simulink model "VFD_final"  (R2025b)
settings: Solver=VariableStepAuto  StartTime=0.0  StopTime=10  RelTol=1e-3
libraries: ee_lib x18, fl_lib x9, nesl_utility x8, eePwmGeneratorTwoLevel x1, dspstat3 x1, eeSinGeneratorThreePhase x1, simulink x1
settings Model: Creator=Administrator  LastModifiedBy=WELCOME
settings SolverCC: AlgebraicLoopSolver=TrustRegion
settings DebuggingCC: UnconnectedInputMsg=warning  UnconnectedOutputMsg=warning  UnconnectedLineMsg=warning
settings ModelReferenceCC: EnableRefExpFcnMdlSchedulingChecks=on
settings SFSimCC: CustomCodeUndefinedFunction=UseInterfaceOnly
settings RTWCC: GPUComputeCapability=3.5  DLArmComputeVersion=19.05

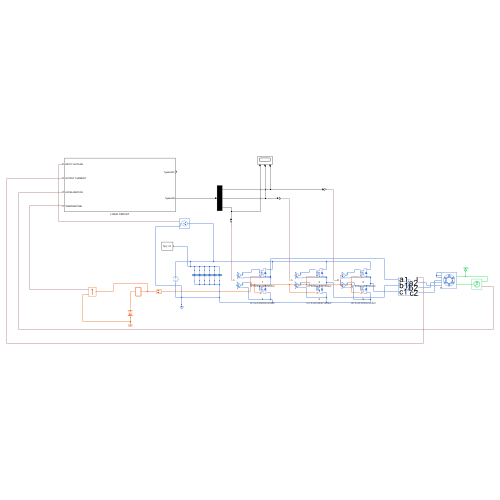
[thumbnail: Simulink's stored preview of the top-level diagram]
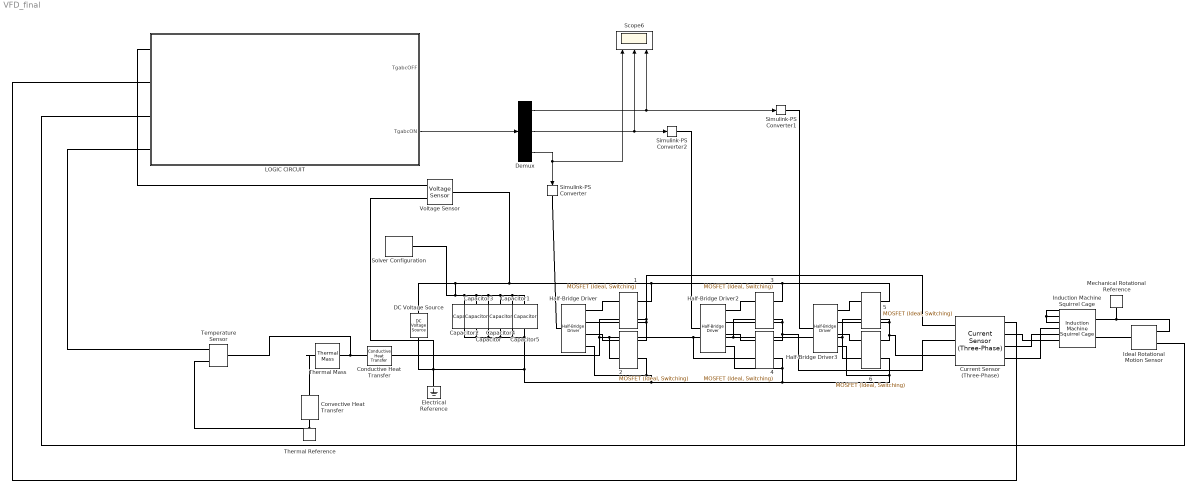
== system VFD_final ==
  {1..6} (6 alike) : ee_lib/Semiconductors & Converters/MOSFET (Ideal, Switching)  PartSpecification="{\"CollectionId\":\"SimscapeElectrical\",\"CollectionVersion\":\"1.0.0\",\"DatasetId\":\"IXYS|IXFN50N120SiC|simscape.electrical.mosfetIdealSwitching\",\"DisplayName\":\"IXYS:IXFN50N120SiC\"}"  port_option=ee.enum.controlport.elec  Rds=0.044 % Datasheet derived Ohm  Goff=2e-09 % Datasheet derived 1/Ohm  Vth=2.6 % Datasheet derived V  diode_param=ee.enum.semiconductors.protectionDiode.nodynamics  diode_Vf=2.21 % Datasheet derived V  diode_Ron=0.015 % Datasheet derived Ohm  diode_Goff=1e-05 % Library default 1/Ohm  diode_C=50e-9 % Parameter not set F  diode_iRM=-235 % Parameter not set A  diode_iF=300 % Parameter not set A  diode_idot=-50 % Parameter not set A/us  diode_trr_param=ee.enum.converters.diodeReverseParam.trr_factor  diode_trr_factor=3 % Parameter not set  diode_trr=15 % Parameter not set us  diode_Qrr=1500 % Parameter not set s*uA  ids_specify=off  ids_priority=None  ids=0 A  ids_nominal_specify=off  ids_nominal_value=1  ids_nominal_unit=A  vds_specify=off  vds_priority=None  vds=0 V  vds_nominal_specify=off  vds_nominal_value=1  vds_nominal_unit=V  vgs_specify=off  vgs_priority=None  vgs=0 V  vgs_nominal_specify=off  vgs_nominal_value=1  vgs_nominal_unit=V  thermal_loss_option=ee.enum.converters.thermalLossOption.tabulated2d  Von_data=[0 0.16 0.32 0.48 0.64 0.81 0.98 1.15 1.33 1.52 1.73 1.93 2.14 2.35 2.59 2.84 3.1 3.35 3.61 3.92 4.24 4.55 4.89 5.23;0 0.29 0.58 0.87 1.16 1.5 1.84 2.18 2.53 2.9 3.28 3.66 4.07 4.5 4.93 5.37 5.8 6.37 6.96 7.55 8.2 8.92 9.63 10.35] % Datasheet derived V  Tj=[25 150] % Datasheet derived degC  Iout_data=[0 4.33 8.67 13 17.34 21.67 26 30.34 34.67 39 43.34 47.67 52.01 56.34 60.67 65.01 69.34 73.68 78.01 82.34 86.68 91.01 95.35 99.68] % Datasheet derived A  Eon_data=[0.11 0.15 0.19 0.22 0.26 0.3 0.34 0.38 0.41 0.45 0.49 0.53 0.56 0.6 0.64 0.68 0.71 0.75 0.79 0.83 0.86 0.9 0.94 0.98 1.01 1.05 1.09 1.13 1.17 1.21 1.25 1.29 1.33 1.38 1.42 1.46 1.5 1.55 1.59 1.63 1.67 1.72 1.76 1.8 1.85 1.9 1.94 1.99 2.04 2.09 2.13 2.18 2.23 2.27 2.32 2.37 2.42 2.46 2.51 2.56 2.6 2.65 2.69 2.74 2.78 2.83 2.87 2.92 2.96 3.01 3.05 3.1] % Datasheet derived mJ  Eoff_data=[0 0.02 0.01 0 0.01 0.02 0.03 0.04 0.05 0.06 0.07 0.08 0.09 0.1 0.11 0.12 0.13 0.14 0.15 0.16 0.17 0.18 0.19 0.2 0.22 0.23 0.24 0.25 0.26 0.27 0.29 0.3 0.31 0.32 0.33 0.34 0.35 0.37 0.38 0.39 0.4 0.41 0.43 0.44 0.45 0.46 0.47 0.48 0.5 0.51 0.52 0.53 0.55 0.56 0.57 0.59 0.6 0.61 0.63 0.64 0.65 0.67 0.68 0.7 0.71 0.73 0.74 0.75 0.77 0.78 0.8 0.81] % Datasheet derived mJ  Eon_data_3D=[zeros(2, 5, 3)] % Parameter not set J  Eoff_data_3D=[zeros(2, 5, 3)] % Parameter not set J  Tj_loss=150 % Datasheet derived degC  Iout_data_loss=[0 1.12 2.23 3.35 4.47 5.58 6.7 7.81 8.93 10.05 11.16 12.28 13.4 14.51 15.63 16.75 17.86 18.98 20.09 21.21 22.33 23.44 24.56 25.68 26.79 27.91 29.02 30.14 31.26 32.37 33.49 34.61 35.72 36.84 37.96 39.07 40.19 41.3 42.42 43.54 44.65 45.77 46.89 48 49.12 50.24 51.35 52.47 53.58 54.7 55.82 56.93 58.05 59.17 60.28 61.4 62.51 63.63 64.75 65.86 66.98 68.1 69.21 70.33 71.45 72.56 73.68 74.79 75.91 77.03 78.14 79.26] % Datasheet derived A  tabulateWithVds=false % Parameter not set  Vds_loss=[0, 150, 300] % Parameter not set V  Eon_scalar=22.86e-3 % Parameter not set J  Eoff_scalar=17.14e-3 % Parameter not set J  Voff=800 % Datasheet derived V  Iout_scalar=600 % Parameter not set A  useCurrentFromPreviousCycle=false % Parameter not set  useVoltageFromPreviousCycle=false % Parameter not set  diodeModelType=ee.enum.converters.diodeModelType.tabulated  diodeTableType=ee.enum.diode.tableType.IfMat  diode_ReverseIVType=ee.enum.diode.diodeReverseIV.constant  diode_IfMat=[0 0.2663 0.5658 2.7227 13.8624 40.5914 79.6704 138.41;0 0.3166 0.63 4.3646 25.9282 65.8936 119.1956 183.5255] % Datasheet derived A  diode_VfMat=[.9, 1.15, 1.25, 1.5, 1.75, 2.17, 2.6, 2.85; .58, .68, .75, 1.1, 1.38, 1.77, 2.27, 2.7] % Parameter not set V  diode_TjVec=[25 150] % Datasheet derived degC  diode_VfVec=[0 1.05 2.1 3.15 4.19 5.24 6.29 7.34] % Datasheet derived V  diode_IfVec=[.1, .2, .5, 1, 2, 4, 7, 10] % Parameter not set A  diode_IrMat=[1e-06, 2e-06, 5e-06, 1e-05, 2.5e-05, 5e-05, .0001; 2e-06, 5e-06, 1e-05, 4e-05, 8e-05, .0002, .0005] % Parameter not set A  diode_VrMat=[10, 100, 200, 250, 300, 325, 350; 10, 70, 160, 220, 270, 300, 320] % Parameter not set V  diode_VrVec=[10, 20, 40, 50, 70, 80, 100] % Parameter not set V  diode_IrVec=[1e-06, 2e-06, 5e-06, 1e-05, 2e-05, 5e-05, .0001] % Parameter not set A  diode_Vr=-600 % Parameter not set V  diode_Ls=150 % Parameter not set nH  diode_Erec=0.03 % Parameter not set J  diode_rec_loss_model=ee.enum.diode.reverseRecoveryModel.fixed  diode_ErecVal=0 % Parameter not set J  diode_scaleWithIandV=true % Parameter not set  diode_ErecMat=zeros(2, 3) % Parameter not set J  diode_TjrecVec=[298.15, 398.15] % Parameter not set K  diode_IfrecVec=[.1, 1, 10] % Parameter not set A  diode_IrecVal=10 % Parameter not set A  diode_VrecVal=10 % Parameter not set V  diode_tFilter=1 / 1000 / 100 % Parameter not set s  separateThermalPortForDiode=false % Parameter not set  thermal_network_parameterization=ee.enum.thermalNetworkTopology.external  Rth=[.03, .2] % Parameter not set K/W  Rth_Cauer=[.03, .1, .2] % Parameter not set K/W  Rth_Foster=[.08, .14, .22, .16] % Parameter not set K/W  thermal_mass_parameterization=ee.enum.thermalNetwork.timeconstant  thermal_mass=[3, 25] % Parameter not set J/K  thermal_mass_Cauer=[3, 10, 25] % Parameter not set J/K  thermal_mass_Foster=[.001, .005, .05, .5] % Parameter not set J/K  thermal_time_constant=[.1, 5] % Parameter not set s  thermal_time_constant_Cauer=[.1, 1, 5] % Parameter not set s  thermal_time_constant_Foster=[7e-05, .0007, .01, .08] % Parameter not set s  thermal_mass_initial_temperatures=[25, 25] % Parameter not set degC  thermal_mass_initial_temperatures_Cauer=[25, 25, 25] % Parameter not set degC  junction_thermal_mass=19.4 % Datasheet derived J/K  Tvec_initial_Foster=[25, 25, 25, 25] % Parameter not set degC  RthDiode=[.03, .2] % Parameter not set K/W  RthCauerDiode=[.03, .1, .2] % Parameter not set K/W  RthFosterDiode=[.03, .2] % Parameter not set K/W  thermalMassDiode=[3, 25] % Parameter not set J/K  thermalMassCauerDiode=[3, 10, 25] % Parameter not set J/K  thermalMassFosterDiode=[33, 50] % Parameter not set J/K  thermalTauDiode=[.1, 5] % Parameter not set s  thermalTauCauerDiode=[.1, 1, 5] % Parameter not set s  thermalTauFosterDiode=[1, 10] % Parameter not set s  thermalMassInitTempDiode=[25, 25] % Parameter not set degC  thermalMassInitTempCauerDiode=[25, 25, 25] % Parameter not set degC  junctionthermalMassDiode=0.1 % Parameter not set J/K  TVecInitialFosterDiode=[25, 25, 25, 25] % Parameter not set degC  no_thermal_network=0 % Parameter not set  mosfet_junction_temperature_specify=off  mosfet_junction_temperature_priority=None  mosfet_junction_temperature=25 degC  mosfet_junction_temperature_nominal_specify=off  mosfet_junction_temperature_nominal_value=1  mosfet_junction_temperature_nominal_unit=degC  diode_junction_temperature_specify=off  diode_junction_temperature_priority=None  diode_junction_temperature=25 degC  diode_junction_temperature_nominal_specify=off  diode_junction_temperature_nominal_value=1  diode_junction_temperature_nominal_unit=degC  Qj_specify=off  Qj_priority=None  Qj=0 W  Qj_nominal_specify=off  Qj_nominal_value=1  Qj_nominal_unit=W  accumulatedSwitchingLosses_specify=off  accumulatedSwitchingLosses_priority=None  accumulatedSwitchingLosses=0 J
      settings: AttributesFormatString=IXYS:IXFN50N120SiC  InternalSimscapePortConfiguration="{\"Bottom\":[],\"Left\":[{\"id\":\"G_elec\",\"label\":\"\",\"type\":\"foundation.electrical.electrical\"},{\"id\":\"H\",\"label\":\"\",\"type\":\"foundation.thermal.thermal\"}],\"Right\":[{\"id\":\"D\",\"label\":\"\",\"type\":\"foundation.electrical.electrical\"},{\"id\":\"S\",\"label\":\"\",\"type\":\"foundation.electrical.electrical\"}],\"Top\":[]}"
  Capacitor{,1..5} (6 alike) : ee_lib/Passive/Capacitor  cap_option=ee.enum.passive.capacitor.capOption.const  c=550e-6 F  Cvec=[1e-05, 1e-06] F  Vvec=[0, 10] V  CV_table_symmetry=ee.enum.passive.capacitor.tableSymmetry.yes  f_vec=[1, 10] kHz  DFext_vec=[.8, 1.2]  enable_C_tol=ee.enum.toleranceApplication.none  averaging_period=0 s  C_tol=5  tol_distribution=ee.enum.toleranceDistribution.uniform  nSigma=4  r=1 Ohm  g=0 1/Ohm  enable_operating_limits=ee.enum.enable.no  operating_limit_action=ee.enum.passive.reportOpLim.warn  max_working_voltage_range=[-25, 25] V  power_rating=1 W  maxTemperature=85 degC  thermalEnable=false  thermalMass=1 J/K  i_specify=off  i_priority=None  i=0 A  i_nominal_specify=off  i_nominal_value=1  i_nominal_unit=A  v_specify=on  v_priority=None  v=565 V  v_nominal_specify=off  v_nominal_value=1  v_nominal_unit=V  vc_specify=off  vc_priority=High  vc=0 V  vc_nominal_specify=off  vc_nominal_value=1  vc_nominal_unit=V  T_specify=off  T_priority=None  T=298.15 K  T_nominal_specify=off  T_nominal_value=1  T_nominal_unit=K
  Conductive Heat Transfer : fl_lib/Thermal/Thermal Elements/Conductive Heat Transfer  thermal_type=foundation.enum.ConstantVariableTabulated.Constant  wall_geometry=foundation.enum.ConductionWallGeometry.Planar  area=20e-4 m^2  thickness=0.3 m  d_in=0.05 m  d_out=0.1 m  L=1 m  th_cond_min=10 W/(K*m)  th_cond=5 W/(K*m)  th_cond_TLU=[413, 401, 392, 383, 371, 357, 342] W/(K*m)  temp_TLU=[200, 273, 400, 600, 800, 1000, 1200] K  T_specify=off  T_priority=None  T=0 K  T_nominal_specify=off  T_nominal_value=1  T_nominal_unit=K  Q_specify=off  Q_priority=None  Q=0 W  Q_nominal_specify=off  Q_nominal_value=1  Q_nominal_unit=W
  Convective Heat Transfer : fl_lib/Thermal/Thermal Elements/Convective Heat Transfer  thermal_type=foundation.enum.constant_variable.constant  area=1e-4 m^2  heat_tr_coeff=20 W/(K*m^2)  min_heat_tr_coeff=1e-3 W/(K*m^2)  T_specify=off  T_priority=None  T=0 K  T_nominal_specify=off  T_nominal_value=1  T_nominal_unit=K  Q_specify=off  Q_priority=None  Q=0 W  Q_nominal_specify=off  Q_nominal_value=1  Q_nominal_unit=W
  Current Sensor (Three-Phase) : ee_lib/Sensors & Transducers/Current Sensor (Three-Phase)
      settings: InternalSimscapePortConfiguration="{\"Bottom\":[],\"Left\":[{\"id\":\"a1\",\"label\":\"a1\",\"type\":\"foundation.electrical.electrical\"},{\"id\":\"b1\",\"label\":\"b1\",\"type\":\"foundation.electrical.electrical\"},{\"id\":\"c1\",\"label\":\"c1\",\"type\":\"foundation.electrical.electrical\"}],\"Right\":[{\"id\":\"I_output\",\"label\":\"I\",\"type\":\"output\"},{\"id\":\"a2\",\"label\":\"a2\",\"type\":\"foundation.electrical.electrical\"},{\"id\":\"b2\",\"label\":\"b2\",\"type\":\"foundation.electrical.electrical\"},{\"id\":\"c2\",\"label\":\"c2\",\"type\":\"foundation.electrical.electrical\"}],\"Top\":[]}"
  DC Voltage Source : ee_lib/Additional Components/SPICE Sources/DC Voltage Source  DC=650 V
  Demux : Demux  Outputs=3
  Electrical Reference : fl_lib/Electrical/Electrical Elements/Electrical Reference
  Half-Bridge Driver : ee_lib/Semiconductors & Converters/Half-Bridge Driver  port_option=ee.enum.controlport.ps  uHigh=2.0 V  uLow=0.8 V  uHighValue=3  uLowValue=0.3  vHigh=22 V  vLow=-3 V  tpLH=50 ns  tdLH=100 ns  tpHL=50 ns  tdHL=100 ns  parameterization=ee.enum.semiconductors.gateDriverParam.outputImpedance  rHigh=2 Ohm  rLow=2 Ohm  tRise=20 ns  tFall=20 ns  cLoad=10 nF  ZonTime_specify=off  ZonTime_priority=None  ZonTime=0 s  ZoffTime_specify=off  ZoffTime_priority=None  ZoffTime=0 s  power_dissipated_high_side_specify=off  power_dissipated_high_side_priority=None  power_dissipated_high_side=0 W  power_dissipated_high_side_nominal_specify=off  power_dissipated_high_side_nominal_value=1  power_dissipated_high_side_nominal_unit=W  power_dissipated_low_side_specify=off  power_dissipated_low_side_priority=None  power_dissipated_low_side=0 W  power_dissipated_low_side_nominal_specify=off  power_dissipated_low_side_nominal_value=1  power_dissipated_low_side_nominal_unit=W
      settings: InternalSimscapePortConfiguration="{\"Bottom\":[],\"Left\":[{\"id\":\"u\",\"label\":\"u\",\"type\":\"input\"}],\"Right\":[{\"id\":\"HO\",\"label\":\"HO\",\"type\":\"foundation.electrical.electrical\"},{\"id\":\"HS\",\"label\":\"HS\",\"type\":\"foundation.electrical.electrical\"},{\"id\":\"LO\",\"label\":\"LO\",\"type\":\"foundation.electrical.electrical\"},{\"id\":\"LS\",\"label\":\"LS\",\"type\":\"foundation.electrical.electrical\"}],\"Top\":[]}"
  Half-Bridge Driver2 : ee_lib/Semiconductors & Converters/Half-Bridge Driver  port_option=ee.enum.controlport.ps  uHigh=2.0 V  uLow=0.8 V  uHighValue=3  uLowValue=0.3  vHigh=22 V  vLow=-3 V  tpLH=50 ns  tdLH=100 ns  tpHL=50 ns  tdHL=100 ns  parameterization=ee.enum.semiconductors.gateDriverParam.outputImpedance  rHigh=2 Ohm  rLow=2 Ohm  tRise=20 ns  tFall=20 ns  cLoad=10 nF  ZonTime_specify=off  ZonTime_priority=None  ZonTime=0 s  ZoffTime_specify=off  ZoffTime_priority=None  ZoffTime=0 s  power_dissipated_high_side_specify=off  power_dissipated_high_side_priority=None  power_dissipated_high_side=0 W  power_dissipated_high_side_nominal_specify=off  power_dissipated_high_side_nominal_value=1  power_dissipated_high_side_nominal_unit=W  power_dissipated_low_side_specify=off  power_dissipated_low_side_priority=None  power_dissipated_low_side=0 W  power_dissipated_low_side_nominal_specify=off  power_dissipated_low_side_nominal_value=1  power_dissipated_low_side_nominal_unit=W
      settings: InternalSimscapePortConfiguration="{\"Bottom\":[],\"Left\":[{\"id\":\"u\",\"label\":\"u\",\"type\":\"input\"}],\"Right\":[{\"id\":\"HO\",\"label\":\"HO\",\"type\":\"foundation.electrical.electrical\"},{\"id\":\"HS\",\"label\":\"HS\",\"type\":\"foundation.electrical.electrical\"},{\"id\":\"LO\",\"label\":\"LO\",\"type\":\"foundation.electrical.electrical\"},{\"id\":\"LS\",\"label\":\"LS\",\"type\":\"foundation.electrical.electrical\"}],\"Top\":[]}"
  Half-Bridge Driver3 : ee_lib/Semiconductors & Converters/Half-Bridge Driver  port_option=ee.enum.controlport.ps  uHigh=2.0 V  uLow=0.8 V  uHighValue=3  uLowValue=0.3  vHigh=22 V  vLow=-3 V  tpLH=50 ns  tdLH=100 ns  tpHL=50 ns  tdHL=100 ns  parameterization=ee.enum.semiconductors.gateDriverParam.outputImpedance  rHigh=2 Ohm  rLow=2 Ohm  tRise=20 ns  tFall=20 ns  cLoad=10 nF  ZonTime_specify=off  ZonTime_priority=None  ZonTime=0 s  ZoffTime_specify=off  ZoffTime_priority=None  ZoffTime=0 s  power_dissipated_high_side_specify=off  power_dissipated_high_side_priority=None  power_dissipated_high_side=0 W  power_dissipated_high_side_nominal_specify=off  power_dissipated_high_side_nominal_value=1  power_dissipated_high_side_nominal_unit=W  power_dissipated_low_side_specify=off  power_dissipated_low_side_priority=None  power_dissipated_low_side=0 W  power_dissipated_low_side_nominal_specify=off  power_dissipated_low_side_nominal_value=1  power_dissipated_low_side_nominal_unit=W
      settings: InternalSimscapePortConfiguration="{\"Bottom\":[],\"Left\":[{\"id\":\"u\",\"label\":\"u\",\"type\":\"input\"}],\"Right\":[{\"id\":\"HO\",\"label\":\"HO\",\"type\":\"foundation.electrical.electrical\"},{\"id\":\"HS\",\"label\":\"HS\",\"type\":\"foundation.electrical.electrical\"},{\"id\":\"LO\",\"label\":\"LO\",\"type\":\"foundation.electrical.electrical\"},{\"id\":\"LS\",\"label\":\"LS\",\"type\":\"foundation.electrical.electrical\"}],\"Top\":[]}"
  Ideal Rotational Motion Sensor : fl_lib/Mechanical/Mechanical Sensors/Ideal Rotational Motion Sensor  reference=foundation.enum.MeasurementReference.difference  acceleration_port=true  velocity_port=false  position_port=false  wrap_angle=false  offset=0 rad
      settings: InternalSimscapePortConfiguration="{\"Bottom\":[],\"Left\":[{\"id\":\"R\",\"label\":\"R\",\"type\":\"foundation.mechanical.rotational.rotational\"}],\"Right\":[{\"id\":\"C\",\"label\":\"C\",\"type\":\"foundation.mechanical.rotational.rotational\"},{\"id\":\"alpha\",\"label\":\"α\",\"type\":\"output\"}],\"Top\":[]}"
  Induction Machine Squirrel Cage : ee_lib/Electromechanical/Asynchronous/Induction Machine Squirrel Cage  port_option=ee.enum.threePhasePort.expanded  SRated=15e3 A*V  VRated=220 V  FRated=60 Hz  nPolePairs=1  param_unit=ee.enum.unit.si  squirrel_cage=ee.enum.squirrelcage.Single  zero_sequence=ee.enum.park.zerosequence.include  initialization_option=ee.enum.asm.initialization.fluxvariables  Rs=0.25 Ohm  Xls=0.4 Ohm  pu_Rs=0.0258  pu_Lls=0.0413  Rrd=0.14 Ohm  Xlrd=0.41 Ohm  pu_Rrd=0.0145  pu_Llrd=0.0424  Rrd1=0.28 Ohm  Xlrd1=0.82 Ohm  Rrd2=0.28 Ohm  Xlrd2=0.82 Ohm  pu_Rrd1=0.0290  pu_Llrd1=0.0848  pu_Rrd2=0.0290  pu_Llrd2=0.0848  Xm=17 Ohm  pu_Lm=1.7562  X0=0.4 Ohm  pu_L0=0.0413  saturation_option=ee.enum.saturation.include  saturation_i=[0, 4, 9, 18, 25, 34, 50, 68, 95, 120] A  saturation_v=[0, 88, 154, 198, 220, 242, 264, 286, 308, 327] V  pu_saturation_i=[0, .176, .396, .792, 1.1, 1.496, 2.2, 2.992, 4.18, 5.28]  pu_saturation_v=[0, .4, .7, .9, 1, 1.1, 1.2, 1.3, 1.4, 1.4864]  connection_option=ee.enum.Connection.delta  angular_position_specify=off  angular_position_priority=None  angular_position=0 deg  angular_position_nominal_specify=off  angular_position_nominal_value=1  angular_position_nominal_unit=deg  pu_psids_specify=off  pu_psids_priority=None  pu_psids=0  pu_psids_nominal_specify=off  pu_psids_nominal_value=1  pu_psids_nominal_unit=1  pu_psiqs_specify=off  pu_psiqs_priority=None  pu_psiqs=0  pu_psiqs_nominal_specify=off  pu_psiqs_nominal_value=1  pu_psiqs_nominal_unit=1  pu_psi0s_specify=off  pu_psi0s_priority=None  pu_psi0s=0  pu_psi0s_nominal_specify=off  pu_psi0s_nominal_value=1  pu_psi0s_nominal_unit=1  pu_psidr_specify=off  pu_psidr_priority=None  pu_psidr=0  pu_psidr_nominal_specify=off  pu_psidr_nominal_value=1  pu_psidr_nominal_unit=1  pu_psiqr_specify=off  pu_psiqr_priority=None  pu_psiqr=0  pu_psiqr_nominal_specify=off  pu_psiqr_nominal_value=1  pu_psiqr_nominal_unit=1  pu_psidr1_specify=off  pu_psidr1_priority=None  pu_psidr1=0  pu_psidr1_nominal_specify=off  pu_psidr1_nominal_value=1  pu_psidr1_nominal_unit=1  pu_psiqr1_specify=off  pu_psiqr1_priority=None  pu_psiqr1=0  pu_psiqr1_nominal_specify=off  pu_psiqr1_nominal_value=1  pu_psiqr1_nominal_unit=1  pu_psidr2_specify=off  pu_psidr2_priority=None  pu_psidr2=0  pu_psidr2_nominal_specify=off  pu_psidr2_nominal_value=1  pu_psidr2_nominal_unit=1  pu_psiqr2_specify=off  pu_psiqr2_priority=None  pu_psiqr2=0  pu_psiqr2_nominal_specify=off  pu_psiqr2_nominal_value=1  pu_psiqr2_nominal_unit=1  psids_specify=off  psids_priority=None  psids=0 Wb  psids_nominal_specify=off  psids_nominal_value=1  psids_nominal_unit=Wb  psiqs_specify=off  psiqs_priority=None  psiqs=0 Wb  psiqs_nominal_specify=off  psiqs_nominal_value=1  psiqs_nominal_unit=Wb  psi0s_specify=off  psi0s_priority=None  psi0s=0 Wb  psi0s_nominal_specify=off  psi0s_nominal_value=1  psi0s_nominal_unit=Wb  psidr_specify=off  psidr_priority=None  psidr=0 Wb  psidr_nominal_specify=off  psidr_nominal_value=1  psidr_nominal_unit=Wb  psiqr_specify=off  psiqr_priority=None  psiqr=0 Wb  psiqr_nominal_specify=off  psiqr_nominal_value=1  psiqr_nominal_unit=Wb  psidr1_specify=off  psidr1_priority=None  psidr1=0 Wb  psidr1_nominal_specify=off  psidr1_nominal_value=1  psidr1_nominal_unit=Wb  psiqr1_specify=off  psiqr1_priority=None  psiqr1=0 Wb  psiqr1_nominal_specify=off  psiqr1_nominal_value=1  psiqr1_nominal_unit=Wb  psidr2_specify=off  psidr2_priority=None  psidr2=0 Wb  psidr2_nominal_specify=off  psidr2_nominal_value=1  psidr2_nominal_unit=Wb  psiqr2_specify=off  psiqr2_priority=None  psiqr2=0 Wb  psiqr2_nominal_specify=off  psiqr2_nominal_value=1  psiqr2_nominal_unit=Wb  slip_specify=off  slip_priority=None  slip=0  slip_nominal_specify=off  slip_nominal_value=1  slip_nominal_unit=1  real_power_generated_specify=off  real_power_generated_priority=None  real_power_generated=0 W  real_power_generated_nominal_specify=off  real_power_generated_nominal_value=1  real_power_generated_nominal_unit=W  mechanical_power_consumed_specify=off  mechanical_power_consumed_priority=None  mechanical_power_consumed=0 W  mechanical_power_consumed_nominal_specify=off  mechanical_power_consumed_nominal_value=1  mechanical_power_consumed_nominal_unit=W  Tmeas=298.15 K  alpha=3.93e-3 1/K  alpha_cage=4.4e-3 1/K  stator_thermal_mass=100 J/K  rotor_thermal_mass=200 J/K  temperatureA_specify=off  temperatureA_priority=High  temperatureA=25 degC  temperatureA_nominal_specify=off  temperatureA_nominal_value=1  temperatureA_nominal_unit=degC  temperatureB_specify=off  temperatureB_priority=High  temperatureB=25 degC  temperatureB_nominal_specify=off  temperatureB_nominal_value=1  temperatureB_nominal_unit=degC  temperatureC_specify=off  temperatureC_priority=High  temperatureC=25 degC  temperatureC_nominal_specify=off  temperatureC_nominal_value=1  temperatureC_nominal_unit=degC  temperatureR_specify=off  temperatureR_priority=High  temperatureR=25 degC  temperatureR_nominal_specify=off  temperatureR_nominal_value=1  temperatureR_nominal_unit=degC
      settings: InternalSimscapePortConfiguration="{\"Bottom\":[],\"Left\":[{\"id\":\"R\",\"label\":\"R\",\"type\":\"foundation.mechanical.rotational.rotational\"},{\"id\":\"C\",\"label\":\"C\",\"type\":\"foundation.mechanical.rotational.rotational\"}],\"Right\":[{\"id\":\"pu_output\",\"label\":\"pu\",\"type\":\"output\"},{\"id\":\"a1\",\"label\":\"a1\",\"type\":\"foundation.electrical.electrical\"},{\"id\":\"b1\",\"label\":\"b1\",\"type\":\"foundation.electrical.electrical\"},{\"id\":\"c1\",\"label\":\"c1\",\"type\":\"foundation.electrical.electrical\"},{\"id\":\"a2\",\"label\":\"a2\",\"type\":\"foundation.electrical.electrical\"},{\"id\":\"b2\",\"label\":\"b2\",\"type\":\"foundation.electrical.electrical\"},{\"id\":\"c2\",\"label\":\"c2\",\"type\":\"foundation.electrical.electrical\"}],\"Top\":[]}"
  LOGIC CIRCUIT : Subsystem
  Mechanical Rotational Reference : fl_lib/Mechanical/Rotational Elements/Mechanical Rotational Reference
  Scope6 : Scope  NumInputPorts=3
      settings: ActiveDisplayYMinimum=1.55591865044998E-5  ActiveDisplayYMaximum=1.5678478245184555E-5  DataLoggingVariableName=ScopeData5
  Simulink-PS Converter : nesl_utility/Simulink-PS Converter  PhysicalDomain=network_engine_domain  SubClassName=ps_input  LeftPortType=input  RightPortType=output  PseudoPeriodic=off  Frequencies=[]  NoiseDistribution=none  NoiseParameters=[]  Unit=1  AffineConversion=off  FilteringAndDerivatives=provide  SimscapeFilterOrder=1  InputFilterTimeConstant=0.001  UdotUserProvided=0
  Simulink-PS Converter1 : nesl_utility/Simulink-PS Converter  PhysicalDomain=network_engine_domain  SubClassName=ps_input  LeftPortType=input  RightPortType=output  PseudoPeriodic=off  Frequencies=[]  NoiseDistribution=none  NoiseParameters=[]  Unit=1  AffineConversion=off  FilteringAndDerivatives=provide  SimscapeFilterOrder=1  InputFilterTimeConstant=0.001  UdotUserProvided=0
  Simulink-PS Converter2 : nesl_utility/Simulink-PS Converter  PhysicalDomain=network_engine_domain  SubClassName=ps_input  LeftPortType=input  RightPortType=output  PseudoPeriodic=off  Frequencies=[]  NoiseDistribution=none  NoiseParameters=[]  Unit=1  AffineConversion=off  FilteringAndDerivatives=provide  SimscapeFilterOrder=1  InputFilterTimeConstant=0.001  UdotUserProvided=0
  Solver Configuration : nesl_utility/Solver Configuration  PhysicalDomain=network_engine_domain  SubClassName=solver  LeftPortType=input  RightPortType=generic  Tones=[]  Harmonics=[]  SimulateNoise=off  Profile=off  UseLocalSampling=off  EnableSwitchedLinearOptims=on  FrequencyDomain=off  UseCCode=off  RelTol=0.001  AbsTol=0.001  MinStep=1e-09  ToWorkspace=off  RevertToSquareIcSolve=off  NumHomotopyIterations=100  PhasorMode=off  PhasorModeNumHarmonics=1  ConsistencySolver=NEWTON_XTOL_AFTER_FTOL  IndexReductionMethod=DerivativeReplacement  DoDC=off  ResidualTolerance=1e-09  ConsistencyTolSource=GLOBAL  ConsistencyAbsTol=0.001  ConsistencyRelTol=0.001  ConsistencyTolFactor=0.01  UseLocalSolver=on  LocalSolverChoice=NE_BACKWARD_EULER_ADVANCER  ResolveIndetEquations=on  FunctionEvalNumThread=1  LocalSolverSampleTime=1e-6  DoFixedCost=off  MaxNonlinIter=3  MaxModeIter=2  ComputeImpulses=off  ImpulseIterations=2  LinearAlgebra=Sparse  LinearAlgebraNumThread=0  EquationFormulation=NE_TIME_EF  DelaysMemoryBudget=1024  AutomaticFiltering=on  FilteringTimeConstant=0.001  PartitionStorageMethod=AS_NEEDED  PartitionMemoryBudget=1024  PartitionMethod=ROBUST  MultibodyUseLocalSolver=off  MultibodyLocalSolverChoice=ODE1  MultibodyLocalSolverSampleTime=0.001
  Temperature Sensor : fl_lib/Thermal/Thermal Sensors/Temperature Sensor  temperature_measure=foundation.enum.MeasurementReference.difference
  Thermal Mass : fl_lib/Thermal/Thermal Elements/Thermal Mass  mass_type=foundation.enum.constant_variable.constant  mass=0.5 kg  sp_heat=900 J/(K*kg)  mass_min=1e-6 kg  num_ports=foundation.enum.numPorts2.two  m_specify=off  m_priority=High  m=1 kg  m_nominal_specify=off  m_nominal_value=1  m_nominal_unit=kg  T_specify=off  T_priority=High  T=300 K  T_nominal_specify=off  T_nominal_value=1  T_nominal_unit=K  Q_specify=off  Q_priority=None  Q=0 W  Q_nominal_specify=off  Q_nominal_value=1  Q_nominal_unit=W
      settings: InternalSimscapePortConfiguration="{\"Bottom\":[],\"Left\":[{\"id\":\"M\",\"label\":\"\",\"type\":\"foundation.thermal.thermal\"}],\"Right\":[{\"id\":\"N\",\"label\":\"\",\"type\":\"foundation.thermal.thermal\"}],\"Top\":[]}"
  Thermal Reference : fl_lib/Thermal/Thermal Elements/Thermal Reference
  Voltage Sensor : fl_lib/Electrical/Electrical Sensors/Voltage Sensor
  wires:
  LOGIC CIRCUIT/2(TgabcON) -> Demux/1
  Demux/1 -> Scope6/3, Simulink-PS Converter1/1
  Demux/2 -> Scope6/2, Simulink-PS Converter2/1
  Demux/3 -> Scope6/1, Simulink-PS Converter/1
  connections:
  DC Voltage Source/LConn1 -- Voltage Sensor/LConn1 -- 1/RConn1 -- 5/RConn1 -- 3/RConn1 -- Solver Configuration/RConn1 -- Capacitor5/LConn1 -- Capacitor1/LConn1 -- Capacitor4/LConn1 -- Capacitor/LConn1 -- Capacitor3/LConn1 -- Capacitor2/LConn1
  5/RConn2 -- 6/RConn1 -- Current Sensor (Three-Phase)/LConn3 -- Half-Bridge Driver3/RConn2
  2/RConn2 -- Half-Bridge Driver/RConn4 -- Half-Bridge Driver2/RConn4 -- 4/RConn2 -- Half-Bridge Driver3/RConn4 -- 6/RConn2 -- Electrical Reference/LConn1 -- Voltage Sensor/RConn2 -- DC Voltage Source/RConn1 -- Capacitor5/RConn1 -- Capacitor3/RConn1 -- Capacitor2/RConn1 -- Capacitor/RConn1 -- Capacitor4/RConn1 -- Capacitor1/RConn1
  Simulink-PS Converter2/RConn1 -- Half-Bridge Driver2/LConn1
  Half-Bridge Driver/RConn1 -- 1/LConn1
  Simulink-PS Converter/RConn1 -- Half-Bridge Driver/LConn1
  6/LConn1 -- Half-Bridge Driver3/RConn3
  Half-Bridge Driver/RConn3 -- 2/LConn1
  3/LConn1 -- Half-Bridge Driver2/RConn1
  4/LConn1 -- Half-Bridge Driver2/RConn3
  Simulink-PS Converter1/RConn1 -- Half-Bridge Driver3/LConn1
  5/LConn1 -- Half-Bridge Driver3/RConn1
  Induction Machine Squirrel Cage/RConn6 -- Induction Machine Squirrel Cage/RConn5 -- Induction Machine Squirrel Cage/RConn7
  3/RConn2 -- Half-Bridge Driver2/RConn2 -- 4/RConn1 -- Current Sensor (Three-Phase)/LConn2
  Induction Machine Squirrel Cage/LConn1 -- Ideal Rotational Motion Sensor/LConn1
  Ideal Rotational Motion Sensor/RConn1 -- Mechanical Rotational Reference/LConn1 -- Induction Machine Squirrel Cage/LConn2
  Induction Machine Squirrel Cage/RConn4 -- Current Sensor (Three-Phase)/RConn4
  Current Sensor (Three-Phase)/RConn3 -- Induction Machine Squirrel Cage/RConn3
  Current Sensor (Three-Phase)/RConn2 -- Induction Machine Squirrel Cage/RConn2
  Half-Bridge Driver/RConn2 -- Current Sensor (Three-Phase)/LConn1 -- 1/RConn2 -- 2/RConn1
  1/LConn2 -- 6/LConn2 -- 5/LConn2 -- 3/LConn2 -- 4/LConn2 -- 2/LConn2 -- Conductive Heat Transfer/LConn1
  Thermal Mass/LConn1 -- Temperature Sensor/LConn1 -- Conductive Heat Transfer/RConn1
  Thermal Mass/RConn1 -- Convective Heat Transfer/LConn1
  Convective Heat Transfer/RConn1 -- Temperature Sensor/RConn1 -- Thermal Reference/LConn1
  Voltage Sensor/RConn1 -- LOGIC CIRCUIT/LConn1
  Current Sensor (Three-Phase)/RConn1 -- LOGIC CIRCUIT/LConn2
  LOGIC CIRCUIT/LConn3 -- Ideal Rotational Motion Sensor/RConn2
  LOGIC CIRCUIT/LConn4 -- Temperature Sensor/RConn2

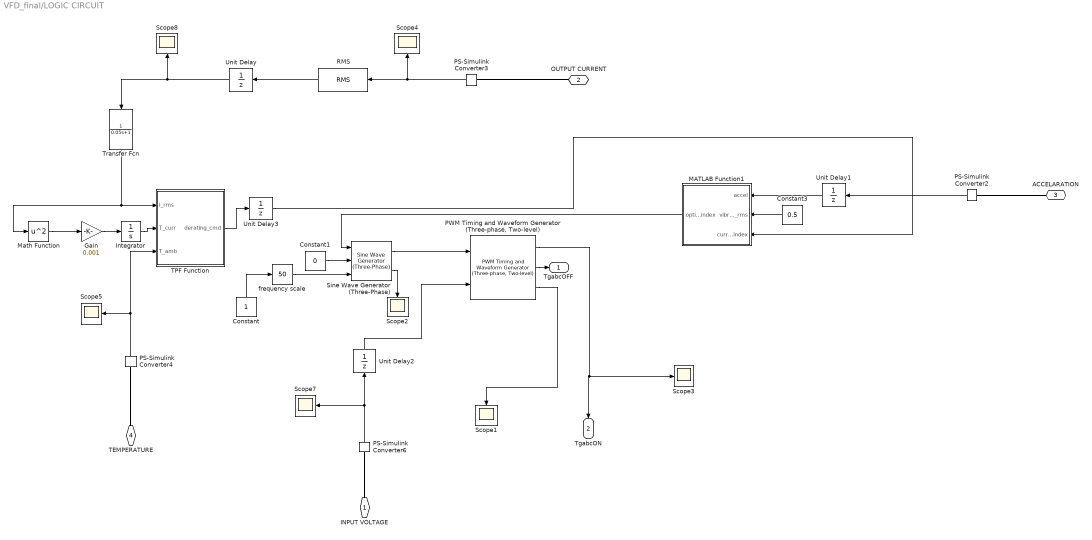
== system VFD_final/LOGIC CIRCUIT ==
  Constant : Constant  SampleTime=1e-6
  Constant1 : Constant  Value=0  SampleTime=1e-6
  Constant3 : Constant  Value=0.5
  Gain : Gain  Gain=0.001
  Integrator : Integrator  InitialCondition=25  LimitOutput=on  UpperSaturationLimit=100  LowerSaturationLimit=25
  MATLAB Function1 : MATLAB Function  TreatAsAtomicUnit=on
  Math Function : Math  Operator=square
  PS-Simulink Converter{2..4,6} (4 alike) : nesl_utility/PS-Simulink Converter  PhysicalDomain=network_engine_domain  SubClassName=ps_output  LeftPortType=input  RightPortType=output  PseudoPeriodic=off  Frequencies=[]  VectorFormat=inherit  Unit=inherit  AffineConversion=off
  "PWM Timing and Waveform Generator (Three-phase, Two-level)" : eePwmGeneratorTwoLevel/PWM Timing and Waveform Generator (Three-phase, Two-level)  PWMMode=Continuous PWM (CPWM)  CPWMMode=SVM: space vector modulation  DPWMMode=60 DPWM (-30 degree shift): -30 degree shift from 60 DPWM  fsw=16000
      settings: SamplingMode=Natural
      settings: LibrarySourceBlock=|
      | ee_sl_lib/Pulse Width
      | Modulation/PWM Timing and Waveform
      | Generator
      | (Three-phase, Two-level)
  RMS : dspstat3/RMS  run=off  directionMode=Each row  dimension=1  InputProcessing=Columns as channels (frame based)  reset_popup=None
  Scope{1..5,7..8} (7 alike) : Scope
      Scope1 settings: ActiveDisplayYMinimum=-0.006381973688274911  ActiveDisplayYMaximum=0.0024847516482319611
      Scope2 settings: ActiveDisplayYMinimum=-0.78539816339718393  ActiveDisplayYMaximum=7.0685834705746577
      Scope3 settings: ActiveDisplayYMinimum=1.5544394651353588E-5  ActiveDisplayYMaximum=1.5696644500548061E-5  DataLoggingVariableName=ScopeData2
      Scope4 settings: ActiveDisplayYMinimum=-4.1578021702740055E-15  ActiveDisplayYMaximum=4.2018297812285585E-15  DataLoggingVariableName=ScopeData3
      Scope5 settings: ActiveDisplayYMinimum=-0.10753529887256302  ActiveDisplayYMaximum=0.20721508094334806  DataLoggingVariableName=ScopeData4
      Scope7 settings: ActiveDisplayYMinimum=85.8621980250673  ActiveDisplayYMaximum=1086.499906431826  DataLoggingVariableName=ScopeData6
      Scope8 settings: ActiveDisplayYMinimum=-4.310238158284335  ActiveDisplayYMaximum=4.7658408295320722  DataLoggingVariableName=ScopeData7
  Sine Wave Generator (Three-Phase) : eeSinGeneratorThreePhase/Sine Wave Generator (Three-Phase)  Ts=1e-6
      settings: LibrarySourceBlock=|
      | ee_sl_lib/General Control/Sine Wave Generator
      | (Three-Phase)
  TPF Function : MATLAB Function  TreatAsAtomicUnit=on
  Transfer Fcn : TransferFcn  Denominator=[0.05 1]
  Unit Delay : UnitDelay  SampleTime=1e-6  HasFrameUpgradeWarning=on
  Unit Delay1 : UnitDelay  SampleTime=1e-6  HasFrameUpgradeWarning=on
  Unit Delay2 : UnitDelay  InitialCondition=600  SampleTime=1e-6  HasFrameUpgradeWarning=on
  Unit Delay3 : UnitDelay  SampleTime=1e-6  HasFrameUpgradeWarning=on
  frequency scale : simulink/Math Operations/Slider Gain  gain=50  low=0  high=100
  INPUT VOLTAGE : PMIOPort  Side=Left
  OUTPUT CURRENT : PMIOPort  Port=2  Side=Left
  ACCELARATION : PMIOPort  Port=3  Side=Left
  TEMPERATURE : PMIOPort  Port=4  Side=Left
  TgabcOFF : Outport
  TgabcON : Outport  Port=2
  wires:
  Sine Wave Generator (Three-Phase)/2 -> Scope2/1
  MATLAB Function1/1(optimal_mod_index) -> Sine Wave Generator (Three-Phase)/1
  Gain/1 -> Integrator/1
  Unit Delay2/1 -> "PWM Timing and Waveform Generator (Three-phase, Two-level)"/2
  Constant1/1 -> Sine Wave Generator (Three-Phase)/2
  Transfer Fcn/1 -> Math Function/1, TPF Function/1(I_rms)
  PS-Simulink Converter3/1 -> Scope4/1, RMS/1
  PS-Simulink Converter4/1 -> TPF Function/3(T_amb), Scope5/1
  Constant3/1 -> MATLAB Function1/2(vibration_rms)
  PS-Simulink Converter2/1 -> Unit Delay1/1
  "PWM Timing and Waveform Generator (Three-phase, Two-level)"/3 -> Scope1/1
  Unit Delay1/1 -> MATLAB Function1/1(accel)
  Integrator/1 -> TPF Function/2(T_curr)
  "PWM Timing and Waveform Generator (Three-phase, Two-level)"/2 -> TgabcOFF/1
  Unit Delay3/1 -> MATLAB Function1/3(current_mod_index)
  TPF Function/1(derating_cmd) -> Unit Delay3/1
  "PWM Timing and Waveform Generator (Three-phase, Two-level)"/1 -> TgabcON/1, Scope3/1
  Unit Delay/1 -> Transfer Fcn/1, Scope8/1
  RMS/1 -> Unit Delay/1
  Sine Wave Generator (Three-Phase)/1 -> "PWM Timing and Waveform Generator (Three-phase, Two-level)"/1
  PS-Simulink Converter6/1 -> Unit Delay2/1, Scope7/1
  Math Function/1 -> Gain/1
  frequency scale/1 -> Sine Wave Generator (Three-Phase)/3
  Constant/1 -> frequency scale/1
  connections:
  OUTPUT CURRENT/RConn1 -- PS-Simulink Converter3/LConn1
  PS-Simulink Converter4/LConn1 -- TEMPERATURE/RConn1
  INPUT VOLTAGE/RConn1 -- PS-Simulink Converter6/LConn1
  PS-Simulink Converter2/LConn1 -- ACCELARATION/RConn1

== matlab function VFD_final/LOGIC CIRCUIT/MATLAB Function1 ==
  data: accel input; optimal_mod_index output; vibration_rms input; current_mod_index input
function optimal_mod_index = POF_Controller(accel, vibration_rms, current_mod_index)
    % Initialize persistent variables for memory across time steps
    persistent best_voltage state wait_timer
    
    % Step size for optimization
    step_size = 0.01;
    
    % Initialize if first run
    if isempty(best_voltage)
        best_voltage = 1.0; 
        state = 0; 
        wait_timer = 0;
    end
    
    % Constants for Hyperloop Logic
    CRUISE_ACCEL = 0.05; 
    MAX_VIBE = 0.5;
    
    % Logic State Machine
    switch state
        case 0 % MONITORING: If cruising at low accel, start reducing voltage for efficiency
            if abs(accel) < CRUISE_ACCEL
                state = 1; 
            else
                best_voltage = 1.0; 
            end
        case 1 % OPTIMIZING: Reduce voltage until vibration becomes too high
            if vibration_rms > MAX_VIBE
                state = 2; 
            else
                best_voltage = best_voltage - step_size; 
            end
        case 2 % RECOVERY: Increase voltage back to safe levels
            best_voltage = best_voltage + 0.05;
            wait_timer = wait_timer + 1;
            if wait_timer > 100
                wait_timer = 0; 
                state = 0; 
            end
        otherwise
            state = 0; % Safety catch-all
    end
    
    % Final Output: Constrain between 0.4 and 1.0
    % We multiply by current_mod_index to ensure it respects the TPF derating
    % Final Output: Constrain between 0.4 and 1.0
    % Multiply by current_mod_index to ensure it respects the TPF derating
    temp_out = best_voltage * current_mod_index; 
    optimal_mod_index = max(min(temp_out, 1.0), 0.4);
end

== matlab function VFD_final/LOGIC CIRCUIT/TPF Function ==
  settings: updateMethod=DISCRETE
  data: I_rms input; derating_cmd output; T_curr input; T_amb input
function derating_cmd = TPF_Controller(I_rms, T_curr, T_amb)
    persistent I_term;
    if isempty(I_term), I_term = 0; end
    
    % Prediction: Heat gain (I^2) vs Cooling (Delta T)
    % Using a small DT for real-time simulation steps
    DT = 0.001; 
    T_pred = T_curr + ((0.05 * I_rms^2) - (0.01 * (T_curr - T_amb))) * DT;
    
    SAFE_LIMIT = 100.0;
    error = SAFE_LIMIT - T_pred;
    
    % PI Derating Logic
    if error < 0 % We are exceeding or about to exceed the limit
        I_term = I_term + (0.01 * error); % Integral action
        output = 1.0 + (0.05 * error) + I_term; 
    else
        I_term = 0; % Reset when safe
        output = 1.0;
    end
    
    % Clamp between 10% (limp home mode) and 100%
    derating_cmd = max(min(output, 1.0), 0.1);
end
